simulink model "g1_walking"  (R2025b)
settings: Solver=daessc  StartTime=0.0  StopTime=4.8  MaxStep=0.0005  RelTol=1e-6  AbsTol=1e-8
model workspace (MAT data in the model file):
  g1_base_p0 = [0; 0; 0.8]
  g1_base_rpy0 = [0; 0; 0]
  g1_command_height = 0.8
  g1_forward_command = 0.1
  g1_gravity = [0 0 -9.81]
  g1_q0 = [-0.05 0 0 -0.05 0 0 0.1 0 0 0 0 0 ... (29 elements, 29x1)]
  g1_qd0 = [0 0 0 0 0 0 0 0 0 0 0 0 ... (29 elements, 29x1)]
  g1_standing = 0
values from neighbouring files (symbols this model uses):
  g1_action_Ts = 0.002    [g1_data.sldd]
  g1_contact_threshold = 1.0    [g1_data.sldd]
  g1_cop_threshold = 5.0    [g1_data.sldd]
  g1_drive_Ts = 0.0005    [g1_data.sldd]
  g1_ground_height = 0.0    [g1_data.sldd]
  g1_limits = -0.87267 -0.2618 -1.0472 -2.5307 -0.5236 -2.7576 -0.087267 -3.0892 -1.5882 -2.618 -1.614429558 -1.972222054 -1.614429558 -0.87267 -0.2618 -1.0472 -2.5307 -2.9671 -2.7576 -0.087267 -3.0892 -2.2515 -2.618 -1.614429558 -1.972222054 -1.614429558 -0.52 -0.52 -2.618 0.5236 0.2618 2.0944 2.8798 2.9671 2.7576 2.8798 2.6704 2.2515 2.618 1.614429558 1.972222054 1.614429558 0.5236 0.2618 2.0944 2.8798 0.5236    [g1_data.sldd]
  g1_tau_max = 50.0 50.0 25.0 88.0 88.0 88.0 139.0 25.0 25.0 25.0 5.0 25.0 5.0 50.0 50.0 25.0 88.0 88.0 88.0 139.0 25.0 25.0 25.0 5.0 25.0 5.0 50.0 50.0 88.0    [g1_data.sldd]
undefined symbols (not defined in the file or in its folder): X, Y, Z
libraries: sm_lib x336, nesl_utility x122, simulink x1
(part 6 of 7)

== system g1_walking/PhysicalPlant/Multibody29/right_hip_roll_link ==
  Inertia : sm_lib/Body Elements/Inertia  InertiaType=Custom  Mass=1.52  MassUnits=kg  CenterOfMass=[0, 0, 0]  CenterOfMassUnits=m  MomentsOfInertia=[0.0023773, 0.0024123, 0.0016595]  MomentsOfInertiaUnits=kg*m^2  ProductsOfInertia=[-1.84e-05, -0.0003908, 3.8e-06]  ProductsOfInertiaUnits=kg*m^2  GraphicType=None  MarkerShape=Inertia  MarkerSize=20  GraphicVisPropType=SimpleVisualProperties  GraphicDiffuseColor=[0.5 0.5 0.5]  GraphicOpacity=1  GraphicSpecularColor=[0.5 0.5 0.5 1.0]  GraphicAmbientColor=[0.15 0.15 0.15 1.0]  GraphicEmissiveColor=[0.0 0.0 0.0 1.0]  GraphicShininess=75
  InertiaOriginTransform : sm_lib/Frames and Transforms/Rigid Transform  RotationMethod=RotationSequence  FollAlignAxisA=+X  BaseAlignAxisA=+Y  FollAlignAxisB=+Y  BaseAlignAxisB=+Z  RotationStandardAxis=+Z  RotationAngle=0  RotationAngleUnits=deg  RotationArbitraryAxis=[0 0 1]  RotationSequenceAxes=BaseAxes  RotationSequence=XYZ  RotationSequenceAngles=[0, 0, 0]  RotationSequenceAnglesUnits=rad  RotationMatrix=[1 0 0;0 1 0;0 0 1]  Quaternion=[1 0 0 0]  TranslationMethod=Cartesian  TranslationCartesianOffset=[0.029812, 0.001045, -0.087934]  TranslationCartesianOffsetUnits=m  TranslationStandardAxis=+Z  TranslationStandardOffset=0  TranslationStandardOffsetUnits=m  TranslationROffset=0  TranslationROffsetUnits=m  TranslationThetaOffset=0  TranslationThetaOffsetUnits=deg  TranslationZOffset=0  TranslationZOffsetUnits=m
  ReferenceFrame : sm_lib/Frames and Transforms/Reference Frame
  Visual : sm_lib/Body Elements/File Solid  ExtGeomFileName=assets/meshes/right_hip_roll_link.STL  UnitType=Custom  ExtGeomFileUnits=m  StepReaderType=HEX  ExportConvexHullGeometry=off  InertiaType=Custom  BasedOnType=DensityFromFile  Density=1000  DensityUnits=kg/m^3  Mass=0  MassUnits=kg  CenterOfMass=[0, 0, 0]  CenterOfMassUnits=m  MomentsOfInertia=[0, 0, 0]  MomentsOfInertiaUnits=kg*m^2  ProductsOfInertia=[0, 0, 0]  ProductsOfInertiaUnits=kg*m^2  GraphicType=FromGeometry  MarkerShape=Sphere  MarkerSize=10  GraphicVisPropType=SimpleVisualProperties  GraphicDiffuseColor=[0.7, 0.7, 0.7]  GraphicOpacity=1  GraphicSpecularColor=[0.5 0.5 0.5 1.0]  GraphicAmbientColor=[0.15 0.15 0.15 1.0]  GraphicEmissiveColor=[0.0 0.0 0.0 1.0]  GraphicShininess=75  DoExposeReferenceFrame=on  SerializedFrames=<Frames/>
  VisualOriginTransform : sm_lib/Frames and Transforms/Rigid Transform  RotationMethod=RotationSequence  FollAlignAxisA=+X  BaseAlignAxisA=+Y  FollAlignAxisB=+Y  BaseAlignAxisB=+Z  RotationStandardAxis=+Z  RotationAngle=0  RotationAngleUnits=deg  RotationArbitraryAxis=[0 0 1]  RotationSequenceAxes=BaseAxes  RotationSequence=XYZ  RotationSequenceAngles=[0, 0, 0]  RotationSequenceAnglesUnits=rad  RotationMatrix=[1 0 0;0 1 0;0 0 1]  Quaternion=[1 0 0 0]  TranslationMethod=Cartesian  TranslationCartesianOffset=[0, 0, 0]  TranslationCartesianOffsetUnits=m  TranslationStandardAxis=+Z  TranslationStandardOffset=0  TranslationStandardOffsetUnits=m  TranslationROffset=0  TranslationROffsetUnits=m  TranslationThetaOffset=0  TranslationThetaOffsetUnits=deg  TranslationZOffset=0  TranslationZOffsetUnits=m
  right_hip_roll_joint_AxisInvTransform : sm_lib/Frames and Transforms/Rigid Transform  RotationMethod=ArbitraryAxis  FollAlignAxisA=+X  BaseAlignAxisA=+Y  FollAlignAxisB=+Y  BaseAlignAxisB=+Z  RotationStandardAxis=+Z  RotationAngle=1.570796326794897  RotationAngleUnits=rad  RotationArbitraryAxis=[-0, 1, 0]  RotationSequenceAxes=FollowerAxes  RotationSequence=XYX  RotationSequenceAngles=[0 0 0]  RotationSequenceAnglesUnits=deg  RotationMatrix=[1 0 0;0 1 0;0 0 1]  Quaternion=[1 0 0 0]  TranslationMethod=Cartesian  TranslationCartesianOffset=[0, 0, 0]  TranslationCartesianOffsetUnits=m  TranslationStandardAxis=+Z  TranslationStandardOffset=0  TranslationStandardOffsetUnits=m  TranslationROffset=0  TranslationROffsetUnits=m  TranslationThetaOffset=0  TranslationThetaOffsetUnits=deg  TranslationZOffset=0  TranslationZOffsetUnits=m
  right_hip_yaw_joint_AxisTransform : sm_lib/Frames and Transforms/Rigid Transform  RotationMethod=ArbitraryAxis  FollAlignAxisA=+X  BaseAlignAxisA=+Y  FollAlignAxisB=+Y  BaseAlignAxisB=+Z  RotationStandardAxis=+Z  RotationAngle=0  RotationAngleUnits=rad  RotationArbitraryAxis=[1, 0, 0]  RotationSequenceAxes=FollowerAxes  RotationSequence=XYX  RotationSequenceAngles=[0 0 0]  RotationSequenceAnglesUnits=deg  RotationMatrix=[1 0 0;0 1 0;0 0 1]  Quaternion=[1 0 0 0]  TranslationMethod=Cartesian  TranslationCartesianOffset=[0, 0, 0]  TranslationCartesianOffsetUnits=m  TranslationStandardAxis=+Z  TranslationStandardOffset=0  TranslationStandardOffsetUnits=m  TranslationROffset=0  TranslationROffsetUnits=m  TranslationThetaOffset=0  TranslationThetaOffsetUnits=deg  TranslationZOffset=0  TranslationZOffsetUnits=m
  right_hip_yaw_joint_OriginTransform : sm_lib/Frames and Transforms/Rigid Transform  RotationMethod=RotationSequence  FollAlignAxisA=+X  BaseAlignAxisA=+Y  FollAlignAxisB=+Y  BaseAlignAxisB=+Z  RotationStandardAxis=+Z  RotationAngle=0  RotationAngleUnits=deg  RotationArbitraryAxis=[0 0 1]  RotationSequenceAxes=BaseAxes  RotationSequence=XYZ  RotationSequenceAngles=[0, 0, 0]  RotationSequenceAnglesUnits=rad  RotationMatrix=[1 0 0;0 1 0;0 0 1]  Quaternion=[1 0 0 0]  TranslationMethod=Cartesian  TranslationCartesianOffset=[0.025001, 0, -0.12412]  TranslationCartesianOffsetUnits=m  TranslationStandardAxis=+Z  TranslationStandardOffset=0  TranslationStandardOffsetUnits=m  TranslationROffset=0  TranslationROffsetUnits=m  TranslationThetaOffset=0  TranslationThetaOffsetUnits=deg  TranslationZOffset=0  TranslationZOffsetUnits=m
  F : PMIOPort  Side=Left
  F1 : PMIOPort  Port=2  Side=Right
  connections:
  Inertia/RConn1 -- InertiaOriginTransform/RConn1
  InertiaOriginTransform/LConn1 -- ReferenceFrame/RConn1 -- VisualOriginTransform/LConn1 -- right_hip_roll_joint_AxisInvTransform/LConn1 -- right_hip_yaw_joint_OriginTransform/LConn1
  Visual/RConn1 -- VisualOriginTransform/RConn1
  right_hip_roll_joint_AxisInvTransform/RConn1 -- F/RConn1
  right_hip_yaw_joint_AxisTransform/RConn1 -- F1/RConn1
  right_hip_yaw_joint_AxisTransform/LConn1 -- right_hip_yaw_joint_OriginTransform/RConn1

== system g1_walking/PhysicalPlant/Multibody29/right_hip_yaw_link ==
  Inertia : sm_lib/Body Elements/Inertia  InertiaType=Custom  Mass=1.702  MassUnits=kg  CenterOfMass=[0, 0, 0]  CenterOfMassUnits=m  MomentsOfInertia=[0.0057774, 0.0076124, 0.003149]  MomentsOfInertiaUnits=kg*m^2  ProductsOfInertia=[0.0007072, -0.0023948, 0.0005411]  ProductsOfInertiaUnits=kg*m^2  GraphicType=None  MarkerShape=Inertia  MarkerSize=20  GraphicVisPropType=SimpleVisualProperties  GraphicDiffuseColor=[0.5 0.5 0.5]  GraphicOpacity=1  GraphicSpecularColor=[0.5 0.5 0.5 1.0]  GraphicAmbientColor=[0.15 0.15 0.15 1.0]  GraphicEmissiveColor=[0.0 0.0 0.0 1.0]  GraphicShininess=75
  InertiaOriginTransform : sm_lib/Frames and Transforms/Rigid Transform  RotationMethod=RotationSequence  FollAlignAxisA=+X  BaseAlignAxisA=+Y  FollAlignAxisB=+Y  BaseAlignAxisB=+Z  RotationStandardAxis=+Z  RotationAngle=0  RotationAngleUnits=deg  RotationArbitraryAxis=[0 0 1]  RotationSequenceAxes=BaseAxes  RotationSequence=XYZ  RotationSequenceAngles=[0, 0, 0]  RotationSequenceAnglesUnits=rad  RotationMatrix=[1 0 0;0 1 0;0 0 1]  Quaternion=[1 0 0 0]  TranslationMethod=Cartesian  TranslationCartesianOffset=[-0.057709, 0.010981, -0.15078]  TranslationCartesianOffsetUnits=m  TranslationStandardAxis=+Z  TranslationStandardOffset=0  TranslationStandardOffsetUnits=m  TranslationROffset=0  TranslationROffsetUnits=m  TranslationThetaOffset=0  TranslationThetaOffsetUnits=deg  TranslationZOffset=0  TranslationZOffsetUnits=m
  ReferenceFrame : sm_lib/Frames and Transforms/Reference Frame
  Visual : sm_lib/Body Elements/File Solid  ExtGeomFileName=assets/meshes/right_hip_yaw_link.STL  UnitType=Custom  ExtGeomFileUnits=m  StepReaderType=HEX  ExportConvexHullGeometry=off  InertiaType=Custom  BasedOnType=DensityFromFile  Density=1000  DensityUnits=kg/m^3  Mass=0  MassUnits=kg  CenterOfMass=[0, 0, 0]  CenterOfMassUnits=m  MomentsOfInertia=[0, 0, 0]  MomentsOfInertiaUnits=kg*m^2  ProductsOfInertia=[0, 0, 0]  ProductsOfInertiaUnits=kg*m^2  GraphicType=FromGeometry  MarkerShape=Sphere  MarkerSize=10  GraphicVisPropType=SimpleVisualProperties  GraphicDiffuseColor=[0.7, 0.7, 0.7]  GraphicOpacity=1  GraphicSpecularColor=[0.5 0.5 0.5 1.0]  GraphicAmbientColor=[0.15 0.15 0.15 1.0]  GraphicEmissiveColor=[0.0 0.0 0.0 1.0]  GraphicShininess=75  DoExposeReferenceFrame=on  SerializedFrames=<Frames/>
  VisualOriginTransform : sm_lib/Frames and Transforms/Rigid Transform  RotationMethod=RotationSequence  FollAlignAxisA=+X  BaseAlignAxisA=+Y  FollAlignAxisB=+Y  BaseAlignAxisB=+Z  RotationStandardAxis=+Z  RotationAngle=0  RotationAngleUnits=deg  RotationArbitraryAxis=[0 0 1]  RotationSequenceAxes=BaseAxes  RotationSequence=XYZ  RotationSequenceAngles=[0, 0, 0]  RotationSequenceAnglesUnits=rad  RotationMatrix=[1 0 0;0 1 0;0 0 1]  Quaternion=[1 0 0 0]  TranslationMethod=Cartesian  TranslationCartesianOffset=[0, 0, 0]  TranslationCartesianOffsetUnits=m  TranslationStandardAxis=+Z  TranslationStandardOffset=0  TranslationStandardOffsetUnits=m  TranslationROffset=0  TranslationROffsetUnits=m  TranslationThetaOffset=0  TranslationThetaOffsetUnits=deg  TranslationZOffset=0  TranslationZOffsetUnits=m
  right_hip_yaw_joint_AxisInvTransform : sm_lib/Frames and Transforms/Rigid Transform  RotationMethod=ArbitraryAxis  FollAlignAxisA=+X  BaseAlignAxisA=+Y  FollAlignAxisB=+Y  BaseAlignAxisB=+Z  RotationStandardAxis=+Z  RotationAngle=0  RotationAngleUnits=rad  RotationArbitraryAxis=[1, 0, 0]  RotationSequenceAxes=FollowerAxes  RotationSequence=XYX  RotationSequenceAngles=[0 0 0]  RotationSequenceAnglesUnits=deg  RotationMatrix=[1 0 0;0 1 0;0 0 1]  Quaternion=[1 0 0 0]  TranslationMethod=Cartesian  TranslationCartesianOffset=[0, 0, 0]  TranslationCartesianOffsetUnits=m  TranslationStandardAxis=+Z  TranslationStandardOffset=0  TranslationStandardOffsetUnits=m  TranslationROffset=0  TranslationROffsetUnits=m  TranslationThetaOffset=0  TranslationThetaOffsetUnits=deg  TranslationZOffset=0  TranslationZOffsetUnits=m
  right_knee_joint_AxisTransform : sm_lib/Frames and Transforms/Rigid Transform  RotationMethod=ArbitraryAxis  FollAlignAxisA=+X  BaseAlignAxisA=+Y  FollAlignAxisB=+Y  BaseAlignAxisB=+Z  RotationStandardAxis=+Z  RotationAngle=1.570796326794897  RotationAngleUnits=rad  RotationArbitraryAxis=[-1, 0, 0]  RotationSequenceAxes=FollowerAxes  RotationSequence=XYX  RotationSequenceAngles=[0 0 0]  RotationSequenceAnglesUnits=deg  RotationMatrix=[1 0 0;0 1 0;0 0 1]  Quaternion=[1 0 0 0]  TranslationMethod=Cartesian  TranslationCartesianOffset=[0, 0, 0]  TranslationCartesianOffsetUnits=m  TranslationStandardAxis=+Z  TranslationStandardOffset=0  TranslationStandardOffsetUnits=m  TranslationROffset=0  TranslationROffsetUnits=m  TranslationThetaOffset=0  TranslationThetaOffsetUnits=deg  TranslationZOffset=0  TranslationZOffsetUnits=m
  right_knee_joint_OriginTransform : sm_lib/Frames and Transforms/Rigid Transform  RotationMethod=RotationSequence  FollAlignAxisA=+X  BaseAlignAxisA=+Y  FollAlignAxisB=+Y  BaseAlignAxisB=+Z  RotationStandardAxis=+Z  RotationAngle=0  RotationAngleUnits=deg  RotationArbitraryAxis=[0 0 1]  RotationSequenceAxes=BaseAxes  RotationSequence=XYZ  RotationSequenceAngles=[0, 0.1749, 0]  RotationSequenceAnglesUnits=rad  RotationMatrix=[1 0 0;0 1 0;0 0 1]  Quaternion=[1 0 0 0]  TranslationMethod=Cartesian  TranslationCartesianOffset=[-0.078273, -0.0021489, -0.17734]  TranslationCartesianOffsetUnits=m  TranslationStandardAxis=+Z  TranslationStandardOffset=0  TranslationStandardOffsetUnits=m  TranslationROffset=0  TranslationROffsetUnits=m  TranslationThetaOffset=0  TranslationThetaOffsetUnits=deg  TranslationZOffset=0  TranslationZOffsetUnits=m
  F : PMIOPort  Side=Left
  F1 : PMIOPort  Port=2  Side=Right
  connections:
  Inertia/RConn1 -- InertiaOriginTransform/RConn1
  InertiaOriginTransform/LConn1 -- ReferenceFrame/RConn1 -- VisualOriginTransform/LConn1 -- right_hip_yaw_joint_AxisInvTransform/LConn1 -- right_knee_joint_OriginTransform/LConn1
  Visual/RConn1 -- VisualOriginTransform/RConn1
  right_hip_yaw_joint_AxisInvTransform/RConn1 -- F/RConn1
  right_knee_joint_AxisTransform/RConn1 -- F1/RConn1
  right_knee_joint_AxisTransform/LConn1 -- right_knee_joint_OriginTransform/RConn1

== system g1_walking/PhysicalPlant/Multibody29/right_knee_link ==
  Inertia : sm_lib/Body Elements/Inertia  InertiaType=Custom  Mass=1.932  MassUnits=kg  CenterOfMass=[0, 0, 0]  CenterOfMassUnits=m  MomentsOfInertia=[0.011329, 0.011277, 0.0015168]  MomentsOfInertiaUnits=kg*m^2  ProductsOfInertia=[0.0007146, 4.49e-05, -4.82e-05]  ProductsOfInertiaUnits=kg*m^2  GraphicType=None  MarkerShape=Inertia  MarkerSize=20  GraphicVisPropType=SimpleVisualProperties  GraphicDiffuseColor=[0.5 0.5 0.5]  GraphicOpacity=1  GraphicSpecularColor=[0.5 0.5 0.5 1.0]  GraphicAmbientColor=[0.15 0.15 0.15 1.0]  GraphicEmissiveColor=[0.0 0.0 0.0 1.0]  GraphicShininess=75
  InertiaOriginTransform : sm_lib/Frames and Transforms/Rigid Transform  RotationMethod=RotationSequence  FollAlignAxisA=+X  BaseAlignAxisA=+Y  FollAlignAxisB=+Y  BaseAlignAxisB=+Z  RotationStandardAxis=+Z  RotationAngle=0  RotationAngleUnits=deg  RotationArbitraryAxis=[0 0 1]  RotationSequenceAxes=BaseAxes  RotationSequence=XYZ  RotationSequenceAngles=[0, 0, 0]  RotationSequenceAnglesUnits=rad  RotationMatrix=[1 0 0;0 1 0;0 0 1]  Quaternion=[1 0 0 0]  TranslationMethod=Cartesian  TranslationCartesianOffset=[0.005457, -0.003964, -0.12074]  TranslationCartesianOffsetUnits=m  TranslationStandardAxis=+Z  TranslationStandardOffset=0  TranslationStandardOffsetUnits=m  TranslationROffset=0  TranslationROffsetUnits=m  TranslationThetaOffset=0  TranslationThetaOffsetUnits=deg  TranslationZOffset=0  TranslationZOffsetUnits=m
  ReferenceFrame : sm_lib/Frames and Transforms/Reference Frame
  Visual : sm_lib/Body Elements/File Solid  ExtGeomFileName=assets/meshes/right_knee_link.STL  UnitType=Custom  ExtGeomFileUnits=m  StepReaderType=HEX  ExportConvexHullGeometry=off  InertiaType=Custom  BasedOnType=DensityFromFile  Density=1000  DensityUnits=kg/m^3  Mass=0  MassUnits=kg  CenterOfMass=[0, 0, 0]  CenterOfMassUnits=m  MomentsOfInertia=[0, 0, 0]  MomentsOfInertiaUnits=kg*m^2  ProductsOfInertia=[0, 0, 0]  ProductsOfInertiaUnits=kg*m^2  GraphicType=FromGeometry  MarkerShape=Sphere  MarkerSize=10  GraphicVisPropType=SimpleVisualProperties  GraphicDiffuseColor=[0.7, 0.7, 0.7]  GraphicOpacity=1  GraphicSpecularColor=[0.5 0.5 0.5 1.0]  GraphicAmbientColor=[0.15 0.15 0.15 1.0]  GraphicEmissiveColor=[0.0 0.0 0.0 1.0]  GraphicShininess=75  DoExposeReferenceFrame=on  SerializedFrames=<Frames/>
  VisualOriginTransform : sm_lib/Frames and Transforms/Rigid Transform  RotationMethod=RotationSequence  FollAlignAxisA=+X  BaseAlignAxisA=+Y  FollAlignAxisB=+Y  BaseAlignAxisB=+Z  RotationStandardAxis=+Z  RotationAngle=0  RotationAngleUnits=deg  RotationArbitraryAxis=[0 0 1]  RotationSequenceAxes=BaseAxes  RotationSequence=XYZ  RotationSequenceAngles=[0, 0, 0]  RotationSequenceAnglesUnits=rad  RotationMatrix=[1 0 0;0 1 0;0 0 1]  Quaternion=[1 0 0 0]  TranslationMethod=Cartesian  TranslationCartesianOffset=[0, 0, 0]  TranslationCartesianOffsetUnits=m  TranslationStandardAxis=+Z  TranslationStandardOffset=0  TranslationStandardOffsetUnits=m  TranslationROffset=0  TranslationROffsetUnits=m  TranslationThetaOffset=0  TranslationThetaOffsetUnits=deg  TranslationZOffset=0  TranslationZOffsetUnits=m
  right_ankle_pitch_joint_AxisTransform : sm_lib/Frames and Transforms/Rigid Transform  RotationMethod=ArbitraryAxis  FollAlignAxisA=+X  BaseAlignAxisA=+Y  FollAlignAxisB=+Y  BaseAlignAxisB=+Z  RotationStandardAxis=+Z  RotationAngle=1.570796326794897  RotationAngleUnits=rad  RotationArbitraryAxis=[-1, 0, 0]  RotationSequenceAxes=FollowerAxes  RotationSequence=XYX  RotationSequenceAngles=[0 0 0]  RotationSequenceAnglesUnits=deg  RotationMatrix=[1 0 0;0 1 0;0 0 1]  Quaternion=[1 0 0 0]  TranslationMethod=Cartesian  TranslationCartesianOffset=[0, 0, 0]  TranslationCartesianOffsetUnits=m  TranslationStandardAxis=+Z  TranslationStandardOffset=0  TranslationStandardOffsetUnits=m  TranslationROffset=0  TranslationROffsetUnits=m  TranslationThetaOffset=0  TranslationThetaOffsetUnits=deg  TranslationZOffset=0  TranslationZOffsetUnits=m
  right_ankle_pitch_joint_OriginTransform : sm_lib/Frames and Transforms/Rigid Transform  RotationMethod=RotationSequence  FollAlignAxisA=+X  BaseAlignAxisA=+Y  FollAlignAxisB=+Y  BaseAlignAxisB=+Z  RotationStandardAxis=+Z  RotationAngle=0  RotationAngleUnits=deg  RotationArbitraryAxis=[0 0 1]  RotationSequenceAxes=BaseAxes  RotationSequence=XYZ  RotationSequenceAngles=[0, 0, 0]  RotationSequenceAnglesUnits=rad  RotationMatrix=[1 0 0;0 1 0;0 0 1]  Quaternion=[1 0 0 0]  TranslationMethod=Cartesian  TranslationCartesianOffset=[0, 9.444499999999999e-05, -0.30001]  TranslationCartesianOffsetUnits=m  TranslationStandardAxis=+Z  TranslationStandardOffset=0  TranslationStandardOffsetUnits=m  TranslationROffset=0  TranslationROffsetUnits=m  TranslationThetaOffset=0  TranslationThetaOffsetUnits=deg  TranslationZOffset=0  TranslationZOffsetUnits=m
  right_knee_joint_AxisInvTransform : sm_lib/Frames and Transforms/Rigid Transform  RotationMethod=ArbitraryAxis  FollAlignAxisA=+X  BaseAlignAxisA=+Y  FollAlignAxisB=+Y  BaseAlignAxisB=+Z  RotationStandardAxis=+Z  RotationAngle=1.570796326794897  RotationAngleUnits=rad  RotationArbitraryAxis=[-1, 0, 0]  RotationSequenceAxes=FollowerAxes  RotationSequence=XYX  RotationSequenceAngles=[0 0 0]  RotationSequenceAnglesUnits=deg  RotationMatrix=[1 0 0;0 1 0;0 0 1]  Quaternion=[1 0 0 0]  TranslationMethod=Cartesian  TranslationCartesianOffset=[0, 0, 0]  TranslationCartesianOffsetUnits=m  TranslationStandardAxis=+Z  TranslationStandardOffset=0  TranslationStandardOffsetUnits=m  TranslationROffset=0  TranslationROffsetUnits=m  TranslationThetaOffset=0  TranslationThetaOffsetUnits=deg  TranslationZOffset=0  TranslationZOffsetUnits=m
  F : PMIOPort  Side=Left
  F1 : PMIOPort  Port=2  Side=Right
  connections:
  Inertia/RConn1 -- InertiaOriginTransform/RConn1
  InertiaOriginTransform/LConn1 -- ReferenceFrame/RConn1 -- VisualOriginTransform/LConn1 -- right_ankle_pitch_joint_OriginTransform/LConn1 -- right_knee_joint_AxisInvTransform/LConn1
  Visual/RConn1 -- VisualOriginTransform/RConn1
  right_ankle_pitch_joint_AxisTransform/RConn1 -- F1/RConn1
  right_ankle_pitch_joint_AxisTransform/LConn1 -- right_ankle_pitch_joint_OriginTransform/RConn1
  right_knee_joint_AxisInvTransform/RConn1 -- F/RConn1

== system g1_walking/PhysicalPlant/Multibody29/right_rubber_hand ==
  Inertia : sm_lib/Body Elements/Inertia  InertiaType=Custom  Mass=0.17  MassUnits=kg  CenterOfMass=[0, 0, 0]  CenterOfMassUnits=m  MomentsOfInertia=[0.00010099485234748, 0.00028135871571621, 0.00021894770413514]  MomentsOfInertiaUnits=kg*m^2  ProductsOfInertia=[-3.30189743286e-06, -7.4301518642e-07, -3.618590790516e-05]  ProductsOfInertiaUnits=kg*m^2  GraphicType=None  MarkerShape=Inertia  MarkerSize=20  GraphicVisPropType=SimpleVisualProperties  GraphicDiffuseColor=[0.5 0.5 0.5]  GraphicOpacity=1  GraphicSpecularColor=[0.5 0.5 0.5 1.0]  GraphicAmbientColor=[0.15 0.15 0.15 1.0]  GraphicEmissiveColor=[0.0 0.0 0.0 1.0]  GraphicShininess=75
  InertiaOriginTransform : sm_lib/Frames and Transforms/Rigid Transform  RotationMethod=RotationSequence  FollAlignAxisA=+X  BaseAlignAxisA=+Y  FollAlignAxisB=+Y  BaseAlignAxisB=+Z  RotationStandardAxis=+Z  RotationAngle=0  RotationAngleUnits=deg  RotationArbitraryAxis=[0 0 1]  RotationSequenceAxes=BaseAxes  RotationSequence=XYZ  RotationSequenceAngles=[0, 0, 0]  RotationSequenceAnglesUnits=rad  RotationMatrix=[1 0 0;0 1 0;0 0 1]  Quaternion=[1 0 0 0]  TranslationMethod=Cartesian  TranslationCartesianOffset=[0.05361310808, 0.0029590524, 0.00215413091]  TranslationCartesianOffsetUnits=m  TranslationStandardAxis=+Z  TranslationStandardOffset=0  TranslationStandardOffsetUnits=m  TranslationROffset=0  TranslationROffsetUnits=m  TranslationThetaOffset=0  TranslationThetaOffsetUnits=deg  TranslationZOffset=0  TranslationZOffsetUnits=m
  ReferenceFrame : sm_lib/Frames and Transforms/Reference Frame
  Visual : sm_lib/Body Elements/File Solid  ExtGeomFileName=assets/meshes/right_rubber_hand.STL  UnitType=Custom  ExtGeomFileUnits=m  StepReaderType=HEX  ExportConvexHullGeometry=off  InertiaType=Custom  BasedOnType=DensityFromFile  Density=1000  DensityUnits=kg/m^3  Mass=0  MassUnits=kg  CenterOfMass=[0, 0, 0]  CenterOfMassUnits=m  MomentsOfInertia=[0, 0, 0]  MomentsOfInertiaUnits=kg*m^2  ProductsOfInertia=[0, 0, 0]  ProductsOfInertiaUnits=kg*m^2  GraphicType=FromGeometry  MarkerShape=Sphere  MarkerSize=10  GraphicVisPropType=SimpleVisualProperties  GraphicDiffuseColor=[0.7, 0.7, 0.7]  GraphicOpacity=1  GraphicSpecularColor=[0.5 0.5 0.5 1.0]  GraphicAmbientColor=[0.15 0.15 0.15 1.0]  GraphicEmissiveColor=[0.0 0.0 0.0 1.0]  GraphicShininess=75  DoExposeReferenceFrame=on  SerializedFrames=<Frames/>
  VisualOriginTransform : sm_lib/Frames and Transforms/Rigid Transform  RotationMethod=RotationSequence  FollAlignAxisA=+X  BaseAlignAxisA=+Y  FollAlignAxisB=+Y  BaseAlignAxisB=+Z  RotationStandardAxis=+Z  RotationAngle=0  RotationAngleUnits=deg  RotationArbitraryAxis=[0 0 1]  RotationSequenceAxes=BaseAxes  RotationSequence=XYZ  RotationSequenceAngles=[0, 0, 0]  RotationSequenceAnglesUnits=rad  RotationMatrix=[1 0 0;0 1 0;0 0 1]  Quaternion=[1 0 0 0]  TranslationMethod=Cartesian  TranslationCartesianOffset=[0, 0, 0]  TranslationCartesianOffsetUnits=m  TranslationStandardAxis=+Z  TranslationStandardOffset=0  TranslationStandardOffsetUnits=m  TranslationROffset=0  TranslationROffsetUnits=m  TranslationThetaOffset=0  TranslationThetaOffsetUnits=deg  TranslationZOffset=0  TranslationZOffsetUnits=m
  F : PMIOPort  Side=Left
  URDFFrame : PMIOPort  Port=2  Side=Right
  connections:
  Inertia/RConn1 -- InertiaOriginTransform/RConn1
  URDFFrame/RConn1 -- ReferenceFrame/RConn1 -- InertiaOriginTransform/LConn1 -- VisualOriginTransform/LConn1 -- F/RConn1
  Visual/RConn1 -- VisualOriginTransform/RConn1

== system g1_walking/PhysicalPlant/Multibody29/right_shoulder_pitch_link ==
  Inertia : sm_lib/Body Elements/Inertia  InertiaType=Custom  Mass=0.718  MassUnits=kg  CenterOfMass=[0, 0, 0]  CenterOfMassUnits=m  MomentsOfInertia=[0.0004291, 0.000453, 0.000423]  MomentsOfInertiaUnits=kg*m^2  ProductsOfInertia=[-2.26e-05, 6.4e-06, 9.2e-06]  ProductsOfInertiaUnits=kg*m^2  GraphicType=None  MarkerShape=Inertia  MarkerSize=20  GraphicVisPropType=SimpleVisualProperties  GraphicDiffuseColor=[0.5 0.5 0.5]  GraphicOpacity=1  GraphicSpecularColor=[0.5 0.5 0.5 1.0]  GraphicAmbientColor=[0.15 0.15 0.15 1.0]  GraphicEmissiveColor=[0.0 0.0 0.0 1.0]  GraphicShininess=75
  InertiaOriginTransform : sm_lib/Frames and Transforms/Rigid Transform  RotationMethod=RotationSequence  FollAlignAxisA=+X  BaseAlignAxisA=+Y  FollAlignAxisB=+Y  BaseAlignAxisB=+Z  RotationStandardAxis=+Z  RotationAngle=0  RotationAngleUnits=deg  RotationArbitraryAxis=[0 0 1]  RotationSequenceAxes=BaseAxes  RotationSequence=XYZ  RotationSequenceAngles=[0, 0, 0]  RotationSequenceAnglesUnits=rad  RotationMatrix=[1 0 0;0 1 0;0 0 1]  Quaternion=[1 0 0 0]  TranslationMethod=Cartesian  TranslationCartesianOffset=[0, -0.035892, -0.011628]  TranslationCartesianOffsetUnits=m  TranslationStandardAxis=+Z  TranslationStandardOffset=0  TranslationStandardOffsetUnits=m  TranslationROffset=0  TranslationROffsetUnits=m  TranslationThetaOffset=0  TranslationThetaOffsetUnits=deg  TranslationZOffset=0  TranslationZOffsetUnits=m
  ReferenceFrame : sm_lib/Frames and Transforms/Reference Frame
  Visual : sm_lib/Body Elements/File Solid  ExtGeomFileName=assets/meshes/right_shoulder_pitch_link.STL  UnitType=Custom  ExtGeomFileUnits=m  StepReaderType=HEX  ExportConvexHullGeometry=off  InertiaType=Custom  BasedOnType=DensityFromFile  Density=1000  DensityUnits=kg/m^3  Mass=0  MassUnits=kg  CenterOfMass=[0, 0, 0]  CenterOfMassUnits=m  MomentsOfInertia=[0, 0, 0]  MomentsOfInertiaUnits=kg*m^2  ProductsOfInertia=[0, 0, 0]  ProductsOfInertiaUnits=kg*m^2  GraphicType=FromGeometry  MarkerShape=Sphere  MarkerSize=10  GraphicVisPropType=SimpleVisualProperties  GraphicDiffuseColor=[0.7, 0.7, 0.7]  GraphicOpacity=1  GraphicSpecularColor=[0.5 0.5 0.5 1.0]  GraphicAmbientColor=[0.15 0.15 0.15 1.0]  GraphicEmissiveColor=[0.0 0.0 0.0 1.0]  GraphicShininess=75  DoExposeReferenceFrame=on  SerializedFrames=<Frames/>
  VisualOriginTransform : sm_lib/Frames and Transforms/Rigid Transform  RotationMethod=RotationSequence  FollAlignAxisA=+X  BaseAlignAxisA=+Y  FollAlignAxisB=+Y  BaseAlignAxisB=+Z  RotationStandardAxis=+Z  RotationAngle=0  RotationAngleUnits=deg  RotationArbitraryAxis=[0 0 1]  RotationSequenceAxes=BaseAxes  RotationSequence=XYZ  RotationSequenceAngles=[0, 0, 0]  RotationSequenceAnglesUnits=rad  RotationMatrix=[1 0 0;0 1 0;0 0 1]  Quaternion=[1 0 0 0]  TranslationMethod=Cartesian  TranslationCartesianOffset=[0, 0, 0]  TranslationCartesianOffsetUnits=m  TranslationStandardAxis=+Z  TranslationStandardOffset=0  TranslationStandardOffsetUnits=m  TranslationROffset=0  TranslationROffsetUnits=m  TranslationThetaOffset=0  TranslationThetaOffsetUnits=deg  TranslationZOffset=0  TranslationZOffsetUnits=m
  right_shoulder_pitch_joint_AxisInvTransform : sm_lib/Frames and Transforms/Rigid Transform  RotationMethod=ArbitraryAxis  FollAlignAxisA=+X  BaseAlignAxisA=+Y  FollAlignAxisB=+Y  BaseAlignAxisB=+Z  RotationStandardAxis=+Z  RotationAngle=1.570796326794897  RotationAngleUnits=rad  RotationArbitraryAxis=[-1, 0, 0]  RotationSequenceAxes=FollowerAxes  RotationSequence=XYX  RotationSequenceAngles=[0 0 0]  RotationSequenceAnglesUnits=deg  RotationMatrix=[1 0 0;0 1 0;0 0 1]  Quaternion=[1 0 0 0]  TranslationMethod=Cartesian  TranslationCartesianOffset=[0, 0, 0]  TranslationCartesianOffsetUnits=m  TranslationStandardAxis=+Z  TranslationStandardOffset=0  TranslationStandardOffsetUnits=m  TranslationROffset=0  TranslationROffsetUnits=m  TranslationThetaOffset=0  TranslationThetaOffsetUnits=deg  TranslationZOffset=0  TranslationZOffsetUnits=m
  right_shoulder_roll_joint_AxisTransform : sm_lib/Frames and Transforms/Rigid Transform  RotationMethod=ArbitraryAxis  FollAlignAxisA=+X  BaseAlignAxisA=+Y  FollAlignAxisB=+Y  BaseAlignAxisB=+Z  RotationStandardAxis=+Z  RotationAngle=1.570796326794897  RotationAngleUnits=rad  RotationArbitraryAxis=[-0, 1, 0]  RotationSequenceAxes=FollowerAxes  RotationSequence=XYX  RotationSequenceAngles=[0 0 0]  RotationSequenceAnglesUnits=deg  RotationMatrix=[1 0 0;0 1 0;0 0 1]  Quaternion=[1 0 0 0]  TranslationMethod=Cartesian  TranslationCartesianOffset=[0, 0, 0]  TranslationCartesianOffsetUnits=m  TranslationStandardAxis=+Z  TranslationStandardOffset=0  TranslationStandardOffsetUnits=m  TranslationROffset=0  TranslationROffsetUnits=m  TranslationThetaOffset=0  TranslationThetaOffsetUnits=deg  TranslationZOffset=0  TranslationZOffsetUnits=m
  right_shoulder_roll_joint_OriginTransform : sm_lib/Frames and Transforms/Rigid Transform  RotationMethod=RotationSequence  FollAlignAxisA=+X  BaseAlignAxisA=+Y  FollAlignAxisB=+Y  BaseAlignAxisB=+Z  RotationStandardAxis=+Z  RotationAngle=0  RotationAngleUnits=deg  RotationArbitraryAxis=[0 0 1]  RotationSequenceAxes=BaseAxes  RotationSequence=XYZ  RotationSequenceAngles=[0.27925, 0, 0]  RotationSequenceAnglesUnits=rad  RotationMatrix=[1 0 0;0 1 0;0 0 1]  Quaternion=[1 0 0 0]  TranslationMethod=Cartesian  TranslationCartesianOffset=[0, -0.038, -0.013831]  TranslationCartesianOffsetUnits=m  TranslationStandardAxis=+Z  TranslationStandardOffset=0  TranslationStandardOffsetUnits=m  TranslationROffset=0  TranslationROffsetUnits=m  TranslationThetaOffset=0  TranslationThetaOffsetUnits=deg  TranslationZOffset=0  TranslationZOffsetUnits=m
  F : PMIOPort  Side=Left
  F1 : PMIOPort  Port=2  Side=Right
  connections:
  Inertia/RConn1 -- InertiaOriginTransform/RConn1
  InertiaOriginTransform/LConn1 -- ReferenceFrame/RConn1 -- VisualOriginTransform/LConn1 -- right_shoulder_pitch_joint_AxisInvTransform/LConn1 -- right_shoulder_roll_joint_OriginTransform/LConn1
  Visual/RConn1 -- VisualOriginTransform/RConn1
  right_shoulder_pitch_joint_AxisInvTransform/RConn1 -- F/RConn1
  right_shoulder_roll_joint_AxisTransform/RConn1 -- F1/RConn1
  right_shoulder_roll_joint_AxisTransform/LConn1 -- right_shoulder_roll_joint_OriginTransform/RConn1

== system g1_walking/PhysicalPlant/Multibody29/right_shoulder_roll_link ==
  Inertia : sm_lib/Body Elements/Inertia  InertiaType=Custom  Mass=0.643  MassUnits=kg  CenterOfMass=[0, 0, 0]  CenterOfMassUnits=m  MomentsOfInertia=[0.0006177, 0.0006912, 0.0003894]  MomentsOfInertiaUnits=kg*m^2  ProductsOfInertia=[5.3e-06, 8.7e-06, 1e-06]  ProductsOfInertiaUnits=kg*m^2  GraphicType=None  MarkerShape=Inertia  MarkerSize=20  GraphicVisPropType=SimpleVisualProperties  GraphicDiffuseColor=[0.5 0.5 0.5]  GraphicOpacity=1  GraphicSpecularColor=[0.5 0.5 0.5 1.0]  GraphicAmbientColor=[0.15 0.15 0.15 1.0]  GraphicEmissiveColor=[0.0 0.0 0.0 1.0]  GraphicShininess=75
  InertiaOriginTransform : sm_lib/Frames and Transforms/Rigid Transform  RotationMethod=RotationSequence  FollAlignAxisA=+X  BaseAlignAxisA=+Y  FollAlignAxisB=+Y  BaseAlignAxisB=+Z  RotationStandardAxis=+Z  RotationAngle=0  RotationAngleUnits=deg  RotationArbitraryAxis=[0 0 1]  RotationSequenceAxes=BaseAxes  RotationSequence=XYZ  RotationSequenceAngles=[0, 0, 0]  RotationSequenceAnglesUnits=rad  RotationMatrix=[1 0 0;0 1 0;0 0 1]  Quaternion=[1 0 0 0]  TranslationMethod=Cartesian  TranslationCartesianOffset=[-0.000227, -0.00727, -0.06324299999999999]  TranslationCartesianOffsetUnits=m  TranslationStandardAxis=+Z  TranslationStandardOffset=0  TranslationStandardOffsetUnits=m  TranslationROffset=0  TranslationROffsetUnits=m  TranslationThetaOffset=0  TranslationThetaOffsetUnits=deg  TranslationZOffset=0  TranslationZOffsetUnits=m
  ReferenceFrame : sm_lib/Frames and Transforms/Reference Frame
  Visual : sm_lib/Body Elements/File Solid  ExtGeomFileName=assets/meshes/right_shoulder_roll_link.STL  UnitType=Custom  ExtGeomFileUnits=m  StepReaderType=HEX  ExportConvexHullGeometry=off  InertiaType=Custom  BasedOnType=DensityFromFile  Density=1000  DensityUnits=kg/m^3  Mass=0  MassUnits=kg  CenterOfMass=[0, 0, 0]  CenterOfMassUnits=m  MomentsOfInertia=[0, 0, 0]  MomentsOfInertiaUnits=kg*m^2  ProductsOfInertia=[0, 0, 0]  ProductsOfInertiaUnits=kg*m^2  GraphicType=FromGeometry  MarkerShape=Sphere  MarkerSize=10  GraphicVisPropType=SimpleVisualProperties  GraphicDiffuseColor=[0.7, 0.7, 0.7]  GraphicOpacity=1  GraphicSpecularColor=[0.5 0.5 0.5 1.0]  GraphicAmbientColor=[0.15 0.15 0.15 1.0]  GraphicEmissiveColor=[0.0 0.0 0.0 1.0]  GraphicShininess=75  DoExposeReferenceFrame=on  SerializedFrames=<Frames/>
  VisualOriginTransform : sm_lib/Frames and Transforms/Rigid Transform  RotationMethod=RotationSequence  FollAlignAxisA=+X  BaseAlignAxisA=+Y  FollAlignAxisB=+Y  BaseAlignAxisB=+Z  RotationStandardAxis=+Z  RotationAngle=0  RotationAngleUnits=deg  RotationArbitraryAxis=[0 0 1]  RotationSequenceAxes=BaseAxes  RotationSequence=XYZ  RotationSequenceAngles=[0, 0, 0]  RotationSequenceAnglesUnits=rad  RotationMatrix=[1 0 0;0 1 0;0 0 1]  Quaternion=[1 0 0 0]  TranslationMethod=Cartesian  TranslationCartesianOffset=[0, 0, 0]  TranslationCartesianOffsetUnits=m  TranslationStandardAxis=+Z  TranslationStandardOffset=0  TranslationStandardOffsetUnits=m  TranslationROffset=0  TranslationROffsetUnits=m  TranslationThetaOffset=0  TranslationThetaOffsetUnits=deg  TranslationZOffset=0  TranslationZOffsetUnits=m
  right_shoulder_roll_joint_AxisInvTransform : sm_lib/Frames and Transforms/Rigid Transform  RotationMethod=ArbitraryAxis  FollAlignAxisA=+X  BaseAlignAxisA=+Y  FollAlignAxisB=+Y  BaseAlignAxisB=+Z  RotationStandardAxis=+Z  RotationAngle=1.570796326794897  RotationAngleUnits=rad  RotationArbitraryAxis=[-0, 1, 0]  RotationSequenceAxes=FollowerAxes  RotationSequence=XYX  RotationSequenceAngles=[0 0 0]  RotationSequenceAnglesUnits=deg  RotationMatrix=[1 0 0;0 1 0;0 0 1]  Quaternion=[1 0 0 0]  TranslationMethod=Cartesian  TranslationCartesianOffset=[0, 0, 0]  TranslationCartesianOffsetUnits=m  TranslationStandardAxis=+Z  TranslationStandardOffset=0  TranslationStandardOffsetUnits=m  TranslationROffset=0  TranslationROffsetUnits=m  TranslationThetaOffset=0  TranslationThetaOffsetUnits=deg  TranslationZOffset=0  TranslationZOffsetUnits=m
  right_shoulder_yaw_joint_AxisTransform : sm_lib/Frames and Transforms/Rigid Transform  RotationMethod=ArbitraryAxis  FollAlignAxisA=+X  BaseAlignAxisA=+Y  FollAlignAxisB=+Y  BaseAlignAxisB=+Z  RotationStandardAxis=+Z  RotationAngle=0  RotationAngleUnits=rad  RotationArbitraryAxis=[1, 0, 0]  RotationSequenceAxes=FollowerAxes  RotationSequence=XYX  RotationSequenceAngles=[0 0 0]  RotationSequenceAnglesUnits=deg  RotationMatrix=[1 0 0;0 1 0;0 0 1]  Quaternion=[1 0 0 0]  TranslationMethod=Cartesian  TranslationCartesianOffset=[0, 0, 0]  TranslationCartesianOffsetUnits=m  TranslationStandardAxis=+Z  TranslationStandardOffset=0  TranslationStandardOffsetUnits=m  TranslationROffset=0  TranslationROffsetUnits=m  TranslationThetaOffset=0  TranslationThetaOffsetUnits=deg  TranslationZOffset=0  TranslationZOffsetUnits=m
  right_shoulder_yaw_joint_OriginTransform : sm_lib/Frames and Transforms/Rigid Transform  RotationMethod=RotationSequence  FollAlignAxisA=+X  BaseAlignAxisA=+Y  FollAlignAxisB=+Y  BaseAlignAxisB=+Z  RotationStandardAxis=+Z  RotationAngle=0  RotationAngleUnits=deg  RotationArbitraryAxis=[0 0 1]  RotationSequenceAxes=BaseAxes  RotationSequence=XYZ  RotationSequenceAngles=[0, 0, 0]  RotationSequenceAnglesUnits=rad  RotationMatrix=[1 0 0;0 1 0;0 0 1]  Quaternion=[1 0 0 0]  TranslationMethod=Cartesian  TranslationCartesianOffset=[0, -0.00624, -0.1032]  TranslationCartesianOffsetUnits=m  TranslationStandardAxis=+Z  TranslationStandardOffset=0  TranslationStandardOffsetUnits=m  TranslationROffset=0  TranslationROffsetUnits=m  TranslationThetaOffset=0  TranslationThetaOffsetUnits=deg  TranslationZOffset=0  TranslationZOffsetUnits=m
  F : PMIOPort  Side=Left
  F1 : PMIOPort  Port=2  Side=Right
  connections:
  Inertia/RConn1 -- InertiaOriginTransform/RConn1
  InertiaOriginTransform/LConn1 -- ReferenceFrame/RConn1 -- VisualOriginTransform/LConn1 -- right_shoulder_roll_joint_AxisInvTransform/LConn1 -- right_shoulder_yaw_joint_OriginTransform/LConn1
  Visual/RConn1 -- VisualOriginTransform/RConn1
  right_shoulder_roll_joint_AxisInvTransform/RConn1 -- F/RConn1
  right_shoulder_yaw_joint_AxisTransform/RConn1 -- F1/RConn1
  right_shoulder_yaw_joint_AxisTransform/LConn1 -- right_shoulder_yaw_joint_OriginTransform/RConn1

== system g1_walking/PhysicalPlant/Multibody29/right_shoulder_yaw_link ==
  Inertia : sm_lib/Body Elements/Inertia  InertiaType=Custom  Mass=0.734  MassUnits=kg  CenterOfMass=[0, 0, 0]  CenterOfMassUnits=m  MomentsOfInertia=[0.0009988, 0.0010605, 0.0004354]  MomentsOfInertiaUnits=kg*m^2  ProductsOfInertia=[2.86e-05, 0.0001412, -7.900000000000001e-06]  ProductsOfInertiaUnits=kg*m^2  GraphicType=None  MarkerShape=Inertia  MarkerSize=20  GraphicVisPropType=SimpleVisualProperties  GraphicDiffuseColor=[0.5 0.5 0.5]  GraphicOpacity=1  GraphicSpecularColor=[0.5 0.5 0.5 1.0]  GraphicAmbientColor=[0.15 0.15 0.15 1.0]  GraphicEmissiveColor=[0.0 0.0 0.0 1.0]  GraphicShininess=75
  InertiaOriginTransform : sm_lib/Frames and Transforms/Rigid Transform  RotationMethod=RotationSequence  FollAlignAxisA=+X  BaseAlignAxisA=+Y  FollAlignAxisB=+Y  BaseAlignAxisB=+Z  RotationStandardAxis=+Z  RotationAngle=0  RotationAngleUnits=deg  RotationArbitraryAxis=[0 0 1]  RotationSequenceAxes=BaseAxes  RotationSequence=XYZ  RotationSequenceAngles=[0, 0, 0]  RotationSequenceAnglesUnits=rad  RotationMatrix=[1 0 0;0 1 0;0 0 1]  Quaternion=[1 0 0 0]  TranslationMethod=Cartesian  TranslationCartesianOffset=[0.010773, 0.002949, -0.072009]  TranslationCartesianOffsetUnits=m  TranslationStandardAxis=+Z  TranslationStandardOffset=0  TranslationStandardOffsetUnits=m  TranslationROffset=0  TranslationROffsetUnits=m  TranslationThetaOffset=0  TranslationThetaOffsetUnits=deg  TranslationZOffset=0  TranslationZOffsetUnits=m
  ReferenceFrame : sm_lib/Frames and Transforms/Reference Frame
  Visual : sm_lib/Body Elements/File Solid  ExtGeomFileName=assets/meshes/right_shoulder_yaw_link.STL  UnitType=Custom  ExtGeomFileUnits=m  StepReaderType=HEX  ExportConvexHullGeometry=off  InertiaType=Custom  BasedOnType=DensityFromFile  Density=1000  DensityUnits=kg/m^3  Mass=0  MassUnits=kg  CenterOfMass=[0, 0, 0]  CenterOfMassUnits=m  MomentsOfInertia=[0, 0, 0]  MomentsOfInertiaUnits=kg*m^2  ProductsOfInertia=[0, 0, 0]  ProductsOfInertiaUnits=kg*m^2  GraphicType=FromGeometry  MarkerShape=Sphere  MarkerSize=10  GraphicVisPropType=SimpleVisualProperties  GraphicDiffuseColor=[0.7, 0.7, 0.7]  GraphicOpacity=1  GraphicSpecularColor=[0.5 0.5 0.5 1.0]  GraphicAmbientColor=[0.15 0.15 0.15 1.0]  GraphicEmissiveColor=[0.0 0.0 0.0 1.0]  GraphicShininess=75  DoExposeReferenceFrame=on  SerializedFrames=<Frames/>
  VisualOriginTransform : sm_lib/Frames and Transforms/Rigid Transform  RotationMethod=RotationSequence  FollAlignAxisA=+X  BaseAlignAxisA=+Y  FollAlignAxisB=+Y  BaseAlignAxisB=+Z  RotationStandardAxis=+Z  RotationAngle=0  RotationAngleUnits=deg  RotationArbitraryAxis=[0 0 1]  RotationSequenceAxes=BaseAxes  RotationSequence=XYZ  RotationSequenceAngles=[0, 0, 0]  RotationSequenceAnglesUnits=rad  RotationMatrix=[1 0 0;0 1 0;0 0 1]  Quaternion=[1 0 0 0]  TranslationMethod=Cartesian  TranslationCartesianOffset=[0, 0, 0]  TranslationCartesianOffsetUnits=m  TranslationStandardAxis=+Z  TranslationStandardOffset=0  TranslationStandardOffsetUnits=m  TranslationROffset=0  TranslationROffsetUnits=m  TranslationThetaOffset=0  TranslationThetaOffsetUnits=deg  TranslationZOffset=0  TranslationZOffsetUnits=m
  right_elbow_joint_AxisTransform : sm_lib/Frames and Transforms/Rigid Transform  RotationMethod=ArbitraryAxis  FollAlignAxisA=+X  BaseAlignAxisA=+Y  FollAlignAxisB=+Y  BaseAlignAxisB=+Z  RotationStandardAxis=+Z  RotationAngle=1.570796326794897  RotationAngleUnits=rad  RotationArbitraryAxis=[-1, 0, 0]  RotationSequenceAxes=FollowerAxes  RotationSequence=XYX  RotationSequenceAngles=[0 0 0]  RotationSequenceAnglesUnits=deg  RotationMatrix=[1 0 0;0 1 0;0 0 1]  Quaternion=[1 0 0 0]  TranslationMethod=Cartesian  TranslationCartesianOffset=[0, 0, 0]  TranslationCartesianOffsetUnits=m  TranslationStandardAxis=+Z  TranslationStandardOffset=0  TranslationStandardOffsetUnits=m  TranslationROffset=0  TranslationROffsetUnits=m  TranslationThetaOffset=0  TranslationThetaOffsetUnits=deg  TranslationZOffset=0  TranslationZOffsetUnits=m
  right_elbow_joint_OriginTransform : sm_lib/Frames and Transforms/Rigid Transform  RotationMethod=RotationSequence  FollAlignAxisA=+X  BaseAlignAxisA=+Y  FollAlignAxisB=+Y  BaseAlignAxisB=+Z  RotationStandardAxis=+Z  RotationAngle=0  RotationAngleUnits=deg  RotationArbitraryAxis=[0 0 1]  RotationSequenceAxes=BaseAxes  RotationSequence=XYZ  RotationSequenceAngles=[0, 0, 0]  RotationSequenceAnglesUnits=rad  RotationMatrix=[1 0 0;0 1 0;0 0 1]  Quaternion=[1 0 0 0]  TranslationMethod=Cartesian  TranslationCartesianOffset=[0.015783, 0, -0.08051800000000001]  TranslationCartesianOffsetUnits=m  TranslationStandardAxis=+Z  TranslationStandardOffset=0  TranslationStandardOffsetUnits=m  TranslationROffset=0  TranslationROffsetUnits=m  TranslationThetaOffset=0  TranslationThetaOffsetUnits=deg  TranslationZOffset=0  TranslationZOffsetUnits=m
  right_shoulder_yaw_joint_AxisInvTransform : sm_lib/Frames and Transforms/Rigid Transform  RotationMethod=ArbitraryAxis  FollAlignAxisA=+X  BaseAlignAxisA=+Y  FollAlignAxisB=+Y  BaseAlignAxisB=+Z  RotationStandardAxis=+Z  RotationAngle=0  RotationAngleUnits=rad  RotationArbitraryAxis=[1, 0, 0]  RotationSequenceAxes=FollowerAxes  RotationSequence=XYX  RotationSequenceAngles=[0 0 0]  RotationSequenceAnglesUnits=deg  RotationMatrix=[1 0 0;0 1 0;0 0 1]  Quaternion=[1 0 0 0]  TranslationMethod=Cartesian  TranslationCartesianOffset=[0, 0, 0]  TranslationCartesianOffsetUnits=m  TranslationStandardAxis=+Z  TranslationStandardOffset=0  TranslationStandardOffsetUnits=m  TranslationROffset=0  TranslationROffsetUnits=m  TranslationThetaOffset=0  TranslationThetaOffsetUnits=deg  TranslationZOffset=0  TranslationZOffsetUnits=m
  F : PMIOPort  Side=Left
  F1 : PMIOPort  Port=2  Side=Right
  connections:
  Inertia/RConn1 -- InertiaOriginTransform/RConn1
  InertiaOriginTransform/LConn1 -- ReferenceFrame/RConn1 -- VisualOriginTransform/LConn1 -- right_elbow_joint_OriginTransform/LConn1 -- right_shoulder_yaw_joint_AxisInvTransform/LConn1
  Visual/RConn1 -- VisualOriginTransform/RConn1
  right_elbow_joint_AxisTransform/RConn1 -- F1/RConn1
  right_elbow_joint_AxisTransform/LConn1 -- right_elbow_joint_OriginTransform/RConn1
  right_shoulder_yaw_joint_AxisInvTransform/RConn1 -- F/RConn1

== system g1_walking/PhysicalPlant/Multibody29/right_wrist_pitch_link ==
  Inertia : sm_lib/Body Elements/Inertia  InertiaType=Custom  Mass=0.48404956  MassUnits=kg  CenterOfMass=[0, 0, 0]  CenterOfMassUnits=m  MomentsOfInertia=[0.00016579646273, 0.0004295405741, 0.00042953697654]  MomentsOfInertiaUnits=kg*m^2  ProductsOfInertia=[-8.1417712e-07, 1.231699194e-05, 1.231206746e-05]  ProductsOfInertiaUnits=kg*m^2  GraphicType=None  MarkerShape=Inertia  MarkerSize=20  GraphicVisPropType=SimpleVisualProperties  GraphicDiffuseColor=[0.5 0.5 0.5]  GraphicOpacity=1  GraphicSpecularColor=[0.5 0.5 0.5 1.0]  GraphicAmbientColor=[0.15 0.15 0.15 1.0]  GraphicEmissiveColor=[0.0 0.0 0.0 1.0]  GraphicShininess=75
  InertiaOriginTransform : sm_lib/Frames and Transforms/Rigid Transform  RotationMethod=RotationSequence  FollAlignAxisA=+X  BaseAlignAxisA=+Y  FollAlignAxisB=+Y  BaseAlignAxisB=+Z  RotationStandardAxis=+Z  RotationAngle=0  RotationAngleUnits=deg  RotationArbitraryAxis=[0 0 1]  RotationSequenceAxes=BaseAxes  RotationSequence=XYZ  RotationSequenceAngles=[0, 0, 0]  RotationSequenceAnglesUnits=rad  RotationMatrix=[1 0 0;0 1 0;0 0 1]  Quaternion=[1 0 0 0]  TranslationMethod=Cartesian  TranslationCartesianOffset=[0.02299989837, 0.00111685314, -0.00111658096]  TranslationCartesianOffsetUnits=m  TranslationStandardAxis=+Z  TranslationStandardOffset=0  TranslationStandardOffsetUnits=m  TranslationROffset=0  TranslationROffsetUnits=m  TranslationThetaOffset=0  TranslationThetaOffsetUnits=deg  TranslationZOffset=0  TranslationZOffsetUnits=m
  ReferenceFrame : sm_lib/Frames and Transforms/Reference Frame
  Visual : sm_lib/Body Elements/File Solid  ExtGeomFileName=assets/meshes/right_wrist_pitch_link.STL  UnitType=Custom  ExtGeomFileUnits=m  StepReaderType=HEX  ExportConvexHullGeometry=off  InertiaType=Custom  BasedOnType=DensityFromFile  Density=1000  DensityUnits=kg/m^3  Mass=0  MassUnits=kg  CenterOfMass=[0, 0, 0]  CenterOfMassUnits=m  MomentsOfInertia=[0, 0, 0]  MomentsOfInertiaUnits=kg*m^2  ProductsOfInertia=[0, 0, 0]  ProductsOfInertiaUnits=kg*m^2  GraphicType=FromGeometry  MarkerShape=Sphere  MarkerSize=10  GraphicVisPropType=SimpleVisualProperties  GraphicDiffuseColor=[0.7, 0.7, 0.7]  GraphicOpacity=1  GraphicSpecularColor=[0.5 0.5 0.5 1.0]  GraphicAmbientColor=[0.15 0.15 0.15 1.0]  GraphicEmissiveColor=[0.0 0.0 0.0 1.0]  GraphicShininess=75  DoExposeReferenceFrame=on  SerializedFrames=<Frames/>
  VisualOriginTransform : sm_lib/Frames and Transforms/Rigid Transform  RotationMethod=RotationSequence  FollAlignAxisA=+X  BaseAlignAxisA=+Y  FollAlignAxisB=+Y  BaseAlignAxisB=+Z  RotationStandardAxis=+Z  RotationAngle=0  RotationAngleUnits=deg  RotationArbitraryAxis=[0 0 1]  RotationSequenceAxes=BaseAxes  RotationSequence=XYZ  RotationSequenceAngles=[0, 0, 0]  RotationSequenceAnglesUnits=rad  RotationMatrix=[1 0 0;0 1 0;0 0 1]  Quaternion=[1 0 0 0]  TranslationMethod=Cartesian  TranslationCartesianOffset=[0, 0, 0]  TranslationCartesianOffsetUnits=m  TranslationStandardAxis=+Z  TranslationStandardOffset=0  TranslationStandardOffsetUnits=m  TranslationROffset=0  TranslationROffsetUnits=m  TranslationThetaOffset=0  TranslationThetaOffsetUnits=deg  TranslationZOffset=0  TranslationZOffsetUnits=m
  right_wrist_pitch_joint_AxisInvTransform : sm_lib/Frames and Transforms/Rigid Transform  RotationMethod=ArbitraryAxis  FollAlignAxisA=+X  BaseAlignAxisA=+Y  FollAlignAxisB=+Y  BaseAlignAxisB=+Z  RotationStandardAxis=+Z  RotationAngle=1.570796326794897  RotationAngleUnits=rad  RotationArbitraryAxis=[-1, 0, 0]  RotationSequenceAxes=FollowerAxes  RotationSequence=XYX  RotationSequenceAngles=[0 0 0]  RotationSequenceAnglesUnits=deg  RotationMatrix=[1 0 0;0 1 0;0 0 1]  Quaternion=[1 0 0 0]  TranslationMethod=Cartesian  TranslationCartesianOffset=[0, 0, 0]  TranslationCartesianOffsetUnits=m  TranslationStandardAxis=+Z  TranslationStandardOffset=0  TranslationStandardOffsetUnits=m  TranslationROffset=0  TranslationROffsetUnits=m  TranslationThetaOffset=0  TranslationThetaOffsetUnits=deg  TranslationZOffset=0  TranslationZOffsetUnits=m
  right_wrist_yaw_joint_AxisTransform : sm_lib/Frames and Transforms/Rigid Transform  RotationMethod=ArbitraryAxis  FollAlignAxisA=+X  BaseAlignAxisA=+Y  FollAlignAxisB=+Y  BaseAlignAxisB=+Z  RotationStandardAxis=+Z  RotationAngle=0  RotationAngleUnits=rad  RotationArbitraryAxis=[1, 0, 0]  RotationSequenceAxes=FollowerAxes  RotationSequence=XYX  RotationSequenceAngles=[0 0 0]  RotationSequenceAnglesUnits=deg  RotationMatrix=[1 0 0;0 1 0;0 0 1]  Quaternion=[1 0 0 0]  TranslationMethod=Cartesian  TranslationCartesianOffset=[0, 0, 0]  TranslationCartesianOffsetUnits=m  TranslationStandardAxis=+Z  TranslationStandardOffset=0  TranslationStandardOffsetUnits=m  TranslationROffset=0  TranslationROffsetUnits=m  TranslationThetaOffset=0  TranslationThetaOffsetUnits=deg  TranslationZOffset=0  TranslationZOffsetUnits=m
  right_wrist_yaw_joint_OriginTransform : sm_lib/Frames and Transforms/Rigid Transform  RotationMethod=RotationSequence  FollAlignAxisA=+X  BaseAlignAxisA=+Y  FollAlignAxisB=+Y  BaseAlignAxisB=+Z  RotationStandardAxis=+Z  RotationAngle=0  RotationAngleUnits=deg  RotationArbitraryAxis=[0 0 1]  RotationSequenceAxes=BaseAxes  RotationSequence=XYZ  RotationSequenceAngles=[0, 0, 0]  RotationSequenceAnglesUnits=rad  RotationMatrix=[1 0 0;0 1 0;0 0 1]  Quaternion=[1 0 0 0]  TranslationMethod=Cartesian  TranslationCartesianOffset=[0.046, 0, 0]  TranslationCartesianOffsetUnits=m  TranslationStandardAxis=+Z  TranslationStandardOffset=0  TranslationStandardOffsetUnits=m  TranslationROffset=0  TranslationROffsetUnits=m  TranslationThetaOffset=0  TranslationThetaOffsetUnits=deg  TranslationZOffset=0  TranslationZOffsetUnits=m
  F : PMIOPort  Side=Left
  F1 : PMIOPort  Port=2  Side=Right
  connections:
  Inertia/RConn1 -- InertiaOriginTransform/RConn1
  InertiaOriginTransform/LConn1 -- ReferenceFrame/RConn1 -- VisualOriginTransform/LConn1 -- right_wrist_pitch_joint_AxisInvTransform/LConn1 -- right_wrist_yaw_joint_OriginTransform/LConn1
  Visual/RConn1 -- VisualOriginTransform/RConn1
  right_wrist_pitch_joint_AxisInvTransform/RConn1 -- F/RConn1
  right_wrist_yaw_joint_AxisTransform/RConn1 -- F1/RConn1
  right_wrist_yaw_joint_AxisTransform/LConn1 -- right_wrist_yaw_joint_OriginTransform/RConn1
